simulink model "sschdlexThreePhaseTwoLevelInverterModel"  (R2026a)
settings: Solver=FixedStepDiscrete  StopTime=0.05
undefined symbols (not defined in the file or in its folder): ee_sli_rtmsupport, gcbh
libraries: fl_lib x17, nesl_utility x17, ee_lib x9
settings Model: DataTypeOverride=Off  Creator=The MathWorks, Inc.  LastModifiedBy=The MathWorks, Inc.
settings OptimizationCC: ConditionallyExecuteInputs=off  InheritOutputTypeSmallerThanSingle=on
settings DebuggingCC: ArtificialAlgebraicLoopMsg=error  SingleTaskRateTransMsg=error
settings HardwareCC: ProdHWDeviceType=ASIC/FPGA->ASIC/FPGA  TargetBitPerLong=64.0  TargetBitPerPointer=64.0  TargetBitPerSizeT=64.0  TargetBitPerPtrDiffT=64.0  TargetLongLongMode=on  TargetIntDivRoundTo=Zero  TargetEndianess=LittleEndian  TargetWordSize=64.0  TargetHWDeviceType=Custom Processor->MATLAB Host Computer  ProdEqTarget=off
settings SimscapeCC: SimscapeNominalValues="[{\"value\":\"1\",\"unit\":\"A\"},{\"value\":\"1\",\"unit\":\"bar\"},{\"value\":\"1\",\"unit\":\"cm^2\"},{\"value\":\"1\",\"unit\":\"cm^3/s\"},{\"value\":\"1\",\"unit\":\"kJ/kg\"},{\"value\":\"1\",\"unit\":\"kW\"},{\"value\":\"1\",\"unit\":\"l\"},{\"value\":\"1\",\"unit\":\"N\"},{\"value\":\"1\",\"unit\":\"N*m\"},{\"value\":\"1\",\"unit\":\"V\"}]"  SimscapeLogType=none  SimscapeLogDataHistory=5000.0

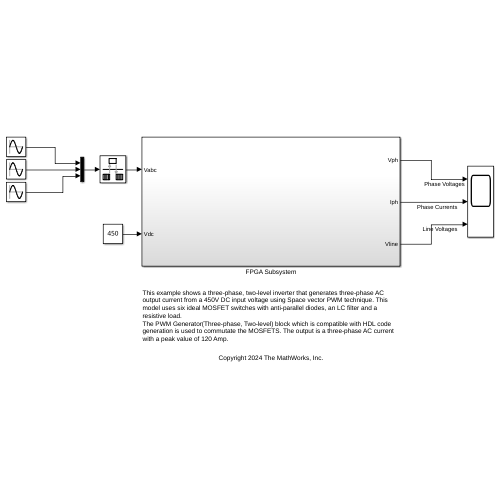
[thumbnail: Simulink's stored preview of the top-level diagram]
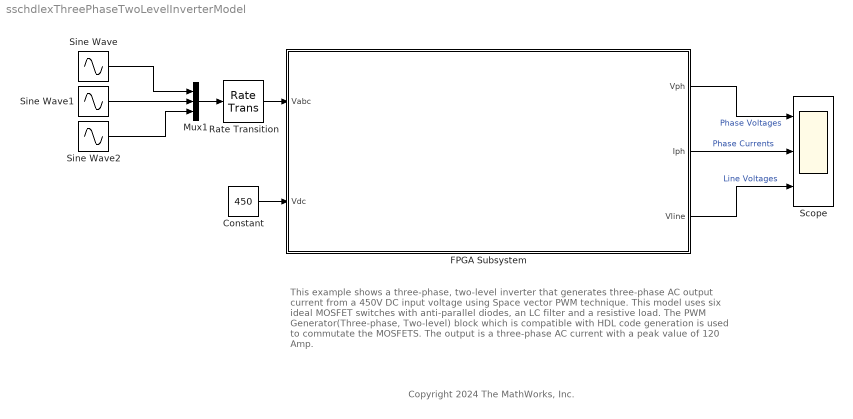
== system sschdlexThreePhaseTwoLevelInverterModel ==
  note: This example shows a three-phase, two-level inverter that generates three-phase AC output current from a 450V DC input voltage using Space vector PWM technique. This model uses six ideal MOSFET switches with anti-parallel diodes, an LC filter and a resistive load.
      | The PWM Generator(Three-phase, Two-level) block which is compatible with HDL code generation is used to commutate the MOSFETS. The output is a three-phase AC current with a peak value of 120 Amp.
  note: Copyright 2024 The MathWorks, Inc.
  Constant : Constant  Value=450  SampleTime=-1
  FPGA Subsystem : Subsystem
  Mux1 : Mux  Inputs=3
  Rate Transition : RateTransition
  Scope : Scope  NumInputPorts=3
      settings: ActiveDisplayYMinimum=159.51111  ActiveDisplayYMaximum=229.40651
  Sine Wave : Sin  Amplitude=200  Frequency=2*pi*50  SampleTime=0
  Sine Wave1 : Sin  Amplitude=200  Frequency=2*pi*50  Phase=-2*pi/3  SampleTime=0
  Sine Wave2 : Sin  Amplitude=200  Frequency=2*pi*50  Phase=-4*pi/3  SampleTime=0
  wires:
  Sine Wave/1 -> Mux1/1
  Sine Wave1/1 -> Mux1/2
  Sine Wave2/1 -> Mux1/3
  Mux1/1 -> Rate Transition/1
  FPGA Subsystem/3(Vline) -> Scope/3  "Line Voltages"
  FPGA Subsystem/1(Vph) -> Scope/1  "Phase Voltages"
  FPGA Subsystem/2(Iph) -> Scope/2  "Phase Currents"
  Rate Transition/1 -> FPGA Subsystem/1(Vabc)
  Constant/1 -> FPGA Subsystem/2(Vdc)

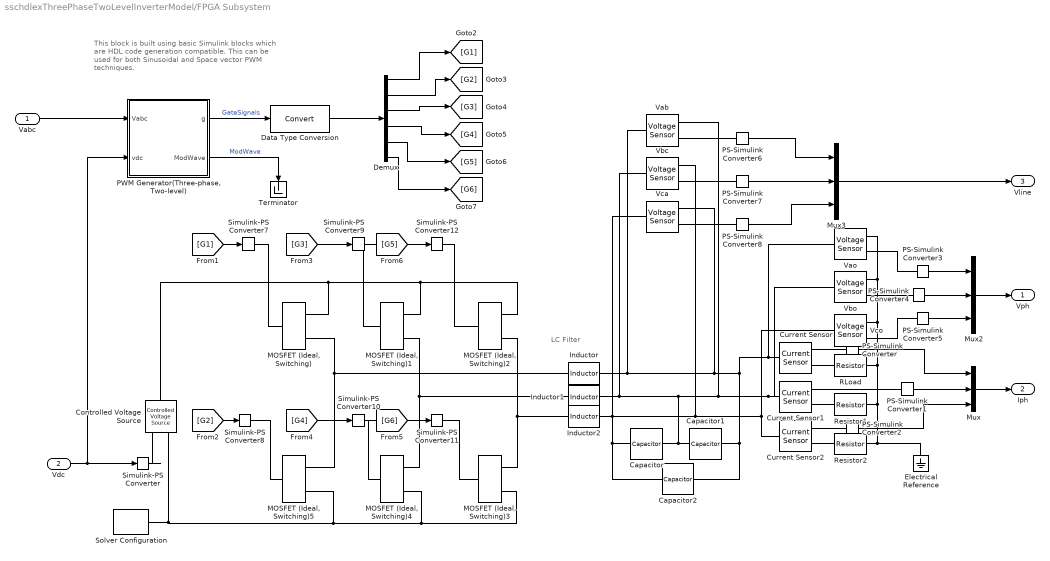
== system sschdlexThreePhaseTwoLevelInverterModel/FPGA Subsystem ==
  note: This block is built using basic Simulink
      | blocks which are HDL code generation
      | compatible. This can be used for both
      | Sinusoidal and Space vector PWM
      | techniques.
  note: LC Filter
  Vabc : Inport
  Vdc : Inport  Port=2
  Capacitor : fl_lib/Electrical/Electrical Elements/Capacitor  c=470e-6 F  r=1e9 Ohm  g=0 1/Ohm  i_specify=off  i_priority=None  i=0 A  i_nominal_specify=off  i_nominal_value=1  i_nominal_unit=A  v_specify=off  v_priority=None  v=0 V  v_nominal_specify=off  v_nominal_value=1  v_nominal_unit=V  vc_specify=off  vc_priority=High  vc=0 V  vc_nominal_specify=off  vc_nominal_value=1  vc_nominal_unit=V
  Capacitor1 : fl_lib/Electrical/Electrical Elements/Capacitor  c=470e-6 F  r=1e9 Ohm  g=0 1/Ohm  i_specify=off  i_priority=None  i=0 A  i_nominal_specify=off  i_nominal_value=1  i_nominal_unit=A  v_specify=off  v_priority=None  v=0 V  v_nominal_specify=off  v_nominal_value=1  v_nominal_unit=V  vc_specify=off  vc_priority=High  vc=0 V  vc_nominal_specify=off  vc_nominal_value=1  vc_nominal_unit=V
  Capacitor2 : fl_lib/Electrical/Electrical Elements/Capacitor  c=470e-6 F  r=1e9 Ohm  g=0 1/Ohm  i_specify=off  i_priority=None  i=0 A  i_nominal_specify=off  i_nominal_value=1  i_nominal_unit=A  v_specify=off  v_priority=None  v=0 V  v_nominal_specify=off  v_nominal_value=1  v_nominal_unit=V  vc_specify=off  vc_priority=High  vc=0 V  vc_nominal_specify=off  vc_nominal_value=1  vc_nominal_unit=V
  Controlled Voltage Source : fl_lib/Electrical/Electrical Sources/Controlled Voltage Source
  Current Sensor : fl_lib/Electrical/Electrical Sensors/Current Sensor
  Current Sensor1 : fl_lib/Electrical/Electrical Sensors/Current Sensor
  Current Sensor2 : fl_lib/Electrical/Electrical Sensors/Current Sensor
  Data Type Conversion : DataTypeConversion  SaturateOnIntegerOverflow=off  RndMeth=Floor
  Demux : Demux  Outputs=6
  Electrical Reference : fl_lib/Electrical/Electrical Elements/Electrical Reference
  Inductor : ee_lib/Passive/Inductor  l=350e-6 H  enable_L_tol=ee.enum.toleranceApplication.none  L_tol=20  tol_distribution=ee.enum.toleranceDistribution.uniform  nSigma=4  r=0 Ohm  g=1e-9 1/Ohm  enable_operating_limits=ee.enum.enable.no  operating_limit_action=ee.enum.passive.reportOpLim.warn  max_working_current=1 A  power_rating=1 W  i_L_specify=off  i_L_priority=High  i_L=0 A  i_L_nominal_specify=off  i_L_nominal_value=1  i_L_nominal_unit=A
  Inductor1 : ee_lib/Passive/Inductor  l=350e-6 H  enable_L_tol=ee.enum.toleranceApplication.none  L_tol=20  tol_distribution=ee.enum.toleranceDistribution.uniform  nSigma=4  r=0 Ohm  g=1e-9 1/Ohm  enable_operating_limits=ee.enum.enable.no  operating_limit_action=ee.enum.passive.reportOpLim.warn  max_working_current=1 A  power_rating=1 W  i_L_specify=off  i_L_priority=High  i_L=0 A  i_L_nominal_specify=off  i_L_nominal_value=1  i_L_nominal_unit=A
  Inductor2 : ee_lib/Passive/Inductor  l=350e-6 H  enable_L_tol=ee.enum.toleranceApplication.none  L_tol=20  tol_distribution=ee.enum.toleranceDistribution.uniform  nSigma=4  r=0 Ohm  g=1e-9 1/Ohm  enable_operating_limits=ee.enum.enable.no  operating_limit_action=ee.enum.passive.reportOpLim.warn  max_working_current=1 A  power_rating=1 W  i_L_specify=off  i_L_priority=High  i_L=0 A  i_L_nominal_specify=off  i_L_nominal_value=1  i_L_nominal_unit=A
  MOSFET (Ideal, Switching){,1..5} (6 alike) : ee_lib/Semiconductors & Converters/MOSFET (Ideal, Switching)  port_option=ee.enum.controlport.ps  Rds=0.001 Ohm  Goff=1e-6 1/Ohm  Vth=0.5 V  diode_param=2  diode_Vf=0.8 V  diode_Ron=0.001 Ohm  diode_Goff=1e-5 1/Ohm  diode_C=50e-9 F  diode_iRM=-235 A  diode_iF=300 A  diode_idot=-50 A/us  diode_trr_param=1  diode_trr_factor=3  diode_trr=15 us  diode_Qrr=1500 s*uA  ids_specify=off  ids_priority=None  ids=0 A  ids_nominal_specify=off  ids_nominal_value=1  ids_nominal_unit=A  vds_specify=off  vds_priority=None  vds=0 V  vds_nominal_specify=off  vds_nominal_value=1  vds_nominal_unit=V  vgs_specify=off  vgs_priority=None  vgs=0 V  vgs_nominal_specify=off  vgs_nominal_value=1  vgs_nominal_unit=V  thermal_loss_option=ee.enum.converters.thermalLossOption.constantvalues  Von_data=[0, 1.8, 3.2, 6, 10, 16; 0, 2, 5.5, 9.5, 15, 25] V  Tj=[298.15, 448.15] K  Iout_data=[0, 20, 40, 60, 80, 100] A  tabulateWithVds=false  Eon_data=[0, 55.04, 124.57, 235.53, 362.12; 0, 71.25, 161.25, 304.88, 468.75] * 1e-6 J  Eoff_data=[0, 18, 30, 56.1, 76.5; 0, 22.5, 37.5, 70.13, 95.63] * 1e-6 J  Eon_data_3D=[zeros(2, 5, 3)] J  Eoff_data_3D=[zeros(2, 5, 3)] J  Tj_loss=[298.15, 448.15] K  Iout_data_loss=[0, 10, 20, 30, 40] A  Vds_loss=[0, 150, 300] V  Eon_scalar=22.86e-3 J  Eoff_scalar=17.14e-3 J  Voff=300 V  Iout_scalar=600 A  useCurrentFromPreviousCycle=false  useVoltageFromPreviousCycle=false  diodeModelType=ee.enum.converters.diodeModelType.pwl  diodeTableType=ee.enum.diode.tableType.IfMat  diode_ReverseIVType=ee.enum.diode.diodeReverseIV.constant  diode_IfMat=[.07, .12, .19, 1.75, 4.24, 7.32, 11.2; .16, .3, .72, 2.14, 4.02, 6.35, 9.12] A  diode_VfMat=[.9, 1.15, 1.25, 1.5, 1.75, 2.17, 2.6, 2.85; .58, .68, .75, 1.1, 1.38, 1.77, 2.27, 2.7] V  diode_TjVec=[25, 125] degC  diode_VfVec=[.5, .7, .9, 1.3, 1.7, 2.1, 2.5] V  diode_IfVec=[.1, .2, .5, 1, 2, 4, 7, 10] A  diode_IrMat=[1e-06, 2e-06, 5e-06, 1e-05, 2.5e-05, 5e-05, .0001; 2e-06, 5e-06, 1e-05, 4e-05, 8e-05, .0002, .0005] A  diode_VrMat=[10, 100, 200, 250, 300, 325, 350; 10, 70, 160, 220, 270, 300, 320] V  diode_VrVec=[10, 20, 40, 50, 70, 80, 100] V  diode_IrVec=[1e-06, 2e-06, 5e-06, 1e-05, 2e-05, 5e-05, .0001] A  diode_Vr=-600 V  diode_Ls=150 nH  diode_Erec=0.03 J  diode_rec_loss_model=ee.enum.diode.reverseRecoveryModel.fixed  diode_ErecVal=0 J  diode_scaleWithIandV=true  diode_ErecMat=zeros(2, 3) J  diodeErecMat3D=zeros(2, 3, 2) J  diode_TjrecVec=[298.15, 398.15] K  diode_IfrecVec=[.1, 1, 10] A  diodeVrecVec=[0, 100] V  diode_IrecVal=10 A  diode_VrecVal=10 V  diode_tFilter=1 / 1000 / 100 s  separateThermalPortForDiode=false  thermal_network_parameterization=ee.enum.thermalNetworkTopology.external  Rth=[.03, .2] K/W  Rth_Cauer=[.03, .1, .2] K/W  Rth_Foster=[.03, .2] K/W  thermal_mass_parameterization=ee.enum.thermalNetwork.timeconstant  thermal_mass=[3, 25] J/K  thermal_mass_Cauer=[3, 10, 25] J/K  thermal_mass_Foster=[33, 50] J/K  thermal_time_constant=[.1, 5] s  thermal_time_constant_Cauer=[.1, 1, 5] s  thermal_time_constant_Foster=[1, 10] s  thermal_mass_initial_temperatures=[25, 25] degC  thermal_mass_initial_temperatures_Cauer=[25, 25, 25] degC  junction_thermal_mass=0.1 J/K  Tvec_initial_Foster=[25, 25, 25, 25] degC  RthDiode=[.03, .2] K/W  RthCauerDiode=[.03, .1, .2] K/W  RthFosterDiode=[.03, .2] K/W  thermalMassDiode=[3, 25] J/K  thermalMassCauerDiode=[3, 10, 25] J/K  thermalMassFosterDiode=[33, 50] J/K  thermalTauDiode=[.1, 5] s  thermalTauCauerDiode=[.1, 1, 5] s  thermalTauFosterDiode=[1, 10] s  thermalMassInitTempDiode=[25, 25] degC  thermalMassInitTempCauerDiode=[25, 25, 25] degC  junctionthermalMassDiode=0.1 J/K  TVecInitialFosterDiode=[25, 25, 25, 25] degC  no_thermal_network=0  mosfet_junction_temperature_specify=off  mosfet_junction_temperature_priority=None  mosfet_junction_temperature=25 degC  mosfet_junction_temperature_nominal_specify=off  mosfet_junction_temperature_nominal_value=1  mosfet_junction_temperature_nominal_unit=degC  diode_junction_temperature_specify=off  diode_junction_temperature_priority=None  diode_junction_temperature=25 degC  diode_junction_temperature_nominal_specify=off  diode_junction_temperature_nominal_value=1  diode_junction_temperature_nominal_unit=degC  Qj_specify=off  Qj_priority=None  Qj=0 W  Qj_nominal_specify=off  Qj_nominal_value=1  Qj_nominal_unit=W  accumulatedSwitchingLosses_specify=off  accumulatedSwitchingLosses_priority=None  accumulatedSwitchingLosses=0 J
  Mux : Mux  Inputs=3
  Mux2 : Mux  Inputs=3
  Mux3 : Mux  Inputs=3
  PS-Simulink Converter{,1..8} (9 alike) : nesl_utility/PS-Simulink Converter  PhysicalDomain=network_engine_domain  SubClassName=ps_output  LeftPortType=input  RightPortType=output  PseudoPeriodic=off  Frequencies=[]  VectorFormat=inherit  Unit=inherit  AffineConversion=off
  "PWM Generator(Three-phase, Two-level)" : Subsystem  LoadFcn=ee_sli_rtmsupport( 'loadfcn', gcbh );  mask(PWM Generator (three-phase, two-level)){PWMMode=Continuous PWM (CPWM), CPWMMode=SVM: space vector modulation, DPWMMode=60 DPWM: 60 degree discontinuous PWM, SamplingMode=Natural, fsw=15e3, Ts=1e-6}
      mask prompts: PWMMode "physmod:ee:library:comments:control:eePwmGeneratorTwoLevel:PWMMode_MP"; CPWMMode "physmod:ee:library:comments:control:eePwmGeneratorTwoLevel:ContinuousPWM_MP"; DPWMMode "physmod:ee:library:comments:control:eePwmGeneratorTwoLevel:DiscontinuousPWM_MP"; SamplingMode "physmod:ee:library:comments:control:eePwmGeneratorTwoLevel:SamplingMode_MP"; fsw "physmod:ee:library:comments:control:eePwmGeneratorTwoLevel:SwitchingFrequencyHz_MP"; Ts "physmod:ee:library:comments:control:eePwmGeneratorTwoLevel:SampleTimes_MP"
      mask help: physmod:ee:library:comments:control:eePwmGeneratorTwoLevel:PWMGeneratorthreephaseTwolevel_MD
      mask init:
      | Tsw = 1/fsw;
      | 
      | if fsw <= 0
      |     error(message('physmod:simscape:compiler:patterns:checks:GreaterThanZero',getString(message('physmod:ee:library:comments:control:eePwmGeneratorTwoLevel:SwitchingFrequencyHz_MP'))));
      | end
      | 
      | if Ts <= 0
      |     error(message('physmod:simscape:compiler:patterns:checks:GreaterThanZero',getString(message('physmod:ee:library:comments:control:eePwmGeneratorTwoLevel:SampleTimes_MP'))));
      | end
      | 
      | if Ts > 1/(10*fsw)
      |     error(message('physmod:simscape:compiler:patterns:checks:LessThanOrEqual',getString(message('physmod:ee:library:comments:control:eePwmGeneratorTwoLevel:SampleTimes_MP')),getString(message('physmod:ee:library:comments:control:eePwmGeneratorTwoLevel:inverseOf10TimesSwitchingFrequency_MP'))));
      | end
      | 
      | switch SamplingMode
      |     case 'Natural'
      |         RateTransitionOnInput = -1;
      |         GateGeneratorX0 = 0;
      |     case 'Asymmetric'
      |         RateTransitionOnInput = 0.5*Tsw;
      |         GateGeneratorX0 = 0.5/fsw;
      |     case 'Symmetric'
      |         RateTransitionOnInput = Tsw;
      |         GateGeneratorX0 = 0;
      | end
      | 
      | 
      | switch PWMMode
      |     case 'Continuous PWM (CPWM)'
      |         switch CPWMMode
      |             case 'SPWM: sinusoidal PWM'
      |                 PWM = 1;
      |             case 'SVM: space vector modulation'
      |                 PWM = 2;
      |         end
      |     case 'Discontinuous PWM (DPWM)'
      |         switch DPWMMode
      |             case '60 DPWM: 60 degree discontinuous PWM'
      |                 PWM = 3;
      |             case '60 DPWM (+30 degree shift): +30 degree shift from 60 DPWM'
      |                 PWM = 4;
      |             case '60 DPWM (-30 degree shift): -30 degree shift from 60 DPWM'
      |                 PWM = 5;
      |             case '30 DPWM: 30 degree discontinuous PWM'
      |                 PWM = 6;
      |             case '120 DPWM: positive dc component'
      |                 PWM = 7;
      |             case '120 DPWM: negative dc component'
      |                 PWM = 8;
      |         end
      | end
      settings: CopyFcn=ee_sli_rtmsupport( 'copyfcn', gcbh );  DeleteFcn=ee_sli_rtmsupport( 'deletefcn', gcbh );  ModelCloseFcn=ee_sli_rtmsupport( 'modelclosefcn', gcbh );  PreSaveFcn=%pe_sli_rtmsupport( 'presavefcn', gcbh );  PostSaveFcn=ee_sli_rtmsupport( 'postsavefcn', gcbh );  PreCopyFcn=ee_sli_rtmsupport( 'precopyfcn', gcbh );  OpenFcn=ee_sli_rtmsupport( 'openfcn', gcbh );  CloseFcn=ee_sli_rtmsupport( 'closefcn', gcbh );  PreDeleteFcn=ee_sli_rtmsupport( 'predeletefcn', gcbh );
      settings: LibrarySourceBlock=|
      | eePwmGeneratorTwoLevel/PWM Generator
      | (Three-phase, Two-level)
      mask Help: web(nesl_help(gcbh))
      mask TypeOptions PWMMode: physmod:ee:library:comments:control:eePwmGeneratorTwoLevel:ContinuousPWMCPWM_PV | physmod:ee:library:comments:control:eePwmGeneratorTwoLevel:DiscontinuousPWMDPWM_PV
      mask Callback PWMMode:
      | switch get_param(gcb,'PWMMode')
      |     case 'Continuous PWM (CPWM)'
      |         set_param(gcb,'MaskVisibilities',{'on';'on';'off';'on';'on';'on'})
      |     case 'Discontinuous PWM (DPWM)'
      |         set_param(gcb,'MaskVisibilities',{'on';'off';'on';'on';'on';'on'})
      | end
      mask TypeOptions CPWMMode: physmod:ee:library:comments:control:eePwmGeneratorTwoLevel:SPWMSinusoidalPWM_PV | physmod:ee:library:comments:control:eePwmGeneratorTwoLevel:SVMSpaceVectorModulation_PV
      mask TypeOptions DPWMMode: physmod:ee:library:comments:control:eePwmGeneratorTwoLevel:x60DPWM60DegreeDiscontinuousPWM_PV | physmod:ee:library:comments:control:eePwmGeneratorTwoLevel:x60DPWM30DegreeShift30DegreeShiftFrom60DPWM_PV | physmod:ee:library:comments:control:eePwmGeneratorTwoLevel:x60DPWM0x2D30DegreeShift0x2D30DegreeShiftFrom60DPWM_PV | physmod:ee:library:comments:control:eePwmGeneratorTwoLevel:x30DPWM30DegreeDiscontinuousPWM_PV | physmod:ee:library:comments:control:eePwmGeneratorTwoLevel:x120DPWMPositiveDcComponent_PV | physmod:ee:library:comments:control:eePwmGeneratorTwoLevel:x120DPWMNegativeDcComponent_PV
      mask TypeOptions SamplingMode: physmod:ee:library:comments:control:eePwmGeneratorTwoLevel:Natural_PV | physmod:ee:library:comments:control:eePwmGeneratorTwoLevel:Asymmetric_PV | physmod:ee:library:comments:control:eePwmGeneratorTwoLevel:Symmetric_PV
      mask DialogControl ParameterGroupVar Prompt: physmod:ee:library:comments:control:eePwmGeneratorTwoLevel:tab_Parameters
      mask DialogControl PWMMode Prompt: PWM mode
      mask DialogControl CPWMMode Prompt: Continuous PWM
      mask DialogControl DPWMMode Prompt: Discontinuous PWM
      mask DialogControl SamplingMode Prompt: Sampling mode
      mask DialogControl fsw Prompt: Switching frequency (Hz)
      mask DialogControl Ts Prompt: Sample time (s)
  RLoad : fl_lib/Electrical/Electrical Elements/Resistor  R=1.65 Ohm  i_specify=off  i_priority=None  i=0 A  i_nominal_specify=off  i_nominal_value=1  i_nominal_unit=A  v_specify=off  v_priority=None  v=0 V  v_nominal_specify=off  v_nominal_value=1  v_nominal_unit=V
  Resistor1 : fl_lib/Electrical/Electrical Elements/Resistor  R=1.65 Ohm  i_specify=off  i_priority=None  i=0 A  i_nominal_specify=off  i_nominal_value=1  i_nominal_unit=A  v_specify=off  v_priority=None  v=0 V  v_nominal_specify=off  v_nominal_value=1  v_nominal_unit=V
  Resistor2 : fl_lib/Electrical/Electrical Elements/Resistor  R=1.65 Ohm  i_specify=off  i_priority=None  i=0 A  i_nominal_specify=off  i_nominal_value=1  i_nominal_unit=A  v_specify=off  v_priority=None  v=0 V  v_nominal_specify=off  v_nominal_value=1  v_nominal_unit=V
  Simulink-PS Converter{,7..12} (7 alike) : nesl_utility/Simulink-PS Converter  PhysicalDomain=network_engine_domain  SubClassName=ps_input  LeftPortType=input  RightPortType=output  PseudoPeriodic=off  Frequencies=[]  NoiseDistribution=none  NoiseParameters=[]  Unit=1  AffineConversion=off  FilteringAndDerivatives=provide  SimscapeFilterOrder=1  InputFilterTimeConstant=0.001  UdotUserProvided=0
  Solver Configuration : nesl_utility/Solver Configuration  PhysicalDomain=network_engine_domain  SubClassName=solver  LeftPortType=input  RightPortType=generic  Tones=[]  Harmonics=[]  SimulateNoise=off  Profile=off  UseLocalSampling=off  EnableSwitchedLinearOptims=on  FrequencyDomain=off  UseCCode=off  RelTol=0.001  AbsTol=0.001  MinStep=1e-09  ToWorkspace=off  RevertToSquareIcSolve=off  NumHomotopyIterations=100  PhasorMode=off  PhasorModeNumHarmonics=1  ConsistencySolver=NEWTON_XTOL_AFTER_FTOL  CanonicalOrdering=UNORDERED  OptimizeIntermediates=UNOPTIMIZED  IndexReductionMethod=DerivativeReplacement  DoDC=off  ResidualTolerance=1e-09  ConsistencyTolSource=GLOBAL  ConsistencyAbsTol=0.001  ConsistencyRelTol=0.001  ConsistencyTolFactor=0.001  UseLocalSolver=on  LocalSolverChoice=NE_BACKWARD_EULER_ADVANCER  ResolveIndetEquations=on  FunctionEvalNumThread=1  LocalSolverSampleTime=1e-6  DoFixedCost=off  MaxNonlinIter=3  MaxModeIter=2  ComputeImpulses=off  ImpulseIterations=2  LinearAlgebra=auto  LinearAlgebraNumThread=0  EquationFormulation=NE_TIME_EF  DelaysMemoryBudget=1024  AutomaticFiltering=on  FilteringTimeConstant=0.001  PartitionStorageMethod=AS_NEEDED  PartitionMemoryBudget=1024  PartitionMethod=ROBUST  MultibodyUseLocalSolver=off  MultibodyLocalSolverChoice=ODE1  MultibodyLocalSolverSampleTime=0.001
  Terminator : Terminator
  Vab : fl_lib/Electrical/Electrical Sensors/Voltage Sensor
  Vao : fl_lib/Electrical/Electrical Sensors/Voltage Sensor
  Vbc : fl_lib/Electrical/Electrical Sensors/Voltage Sensor
  Vbo : fl_lib/Electrical/Electrical Sensors/Voltage Sensor
  Vca : fl_lib/Electrical/Electrical Sensors/Voltage Sensor
  Vco : fl_lib/Electrical/Electrical Sensors/Voltage Sensor
  Vph : Outport
  Iph : Outport  Port=2
  Vline : Outport  Port=3
  wires:
  Demux/2 -> [G2]
  [G5] -> Simulink-PS Converter12/1
  PS-Simulink Converter5/1 -> Mux2/3
  PS-Simulink Converter/1 -> Mux/1
  [G1] -> Simulink-PS Converter7/1
  [G4] -> Simulink-PS Converter10/1
  Demux/3 -> [G3]
  PS-Simulink Converter1/1 -> Mux/2
  Mux/1 -> Iph/1
  Vdc/1 -> Simulink-PS Converter/1, "PWM Generator(Three-phase, Two-level)"/2(vdc)
  [G2] -> Simulink-PS Converter8/1
  PS-Simulink Converter3/1 -> Mux2/1
  Demux/1 -> [G1]
  Data Type Conversion/1 -> Demux/1
  Demux/4 -> [G4]
  Demux/6 -> [G6]
  Demux/5 -> [G5]
  PS-Simulink Converter2/1 -> Mux/3
  [G3] -> Simulink-PS Converter9/1
  "PWM Generator(Three-phase, Two-level)"/1(g) -> Data Type Conversion/1  "GateSignals"
  Mux3/1 -> Vline/1
  PS-Simulink Converter4/1 -> Mux2/2
  Mux2/1 -> Vph/1
  [G6] -> Simulink-PS Converter11/1
  "PWM Generator(Three-phase, Two-level)"/2(ModWave) -> Terminator/1  "ModWave"
  Vabc/1 -> "PWM Generator(Three-phase, Two-level)"/1(Vabc)
  PS-Simulink Converter6/1 -> Mux3/1
  PS-Simulink Converter7/1 -> Mux3/2
  PS-Simulink Converter8/1 -> Mux3/3
  connections:
  Inductor/LConn1 -- "MOSFET (Ideal, Switching)5"/RConn1 -- "MOSFET (Ideal, Switching)"/RConn2
  "MOSFET (Ideal, Switching)2"/RConn1 -- "MOSFET (Ideal, Switching)1"/RConn1 -- "MOSFET (Ideal, Switching)"/RConn1 -- Controlled Voltage Source/LConn1
  Capacitor/LConn1 -- Vco/LConn1 -- Current Sensor2/LConn1 -- Vbc/RConn2 -- Vca/LConn1 -- Inductor2/RConn1 -- Capacitor2/LConn1
  RLoad/LConn1 -- Current Sensor/RConn2
  Resistor2/RConn1 -- Vao/RConn2 -- Vbo/RConn2 -- Vco/RConn2 -- RLoad/RConn1 -- Resistor1/RConn1 -- Electrical Reference/LConn1
  Inductor1/LConn1 -- "MOSFET (Ideal, Switching)4"/RConn1 -- "MOSFET (Ideal, Switching)1"/RConn2
  "MOSFET (Ideal, Switching)3"/RConn2 -- "MOSFET (Ideal, Switching)4"/RConn2 -- "MOSFET (Ideal, Switching)5"/RConn2 -- Solver Configuration/RConn1 -- Controlled Voltage Source/RConn2
  Resistor1/LConn1 -- Current Sensor1/RConn2
  Simulink-PS Converter10/RConn1 -- "MOSFET (Ideal, Switching)4"/LConn1
  Resistor2/LConn1 -- Current Sensor2/RConn2
  Capacitor/RConn1 -- Inductor1/RConn1 -- Vbc/LConn1 -- Vbo/LConn1 -- Current Sensor1/LConn1 -- Vab/RConn2 -- Capacitor1/LConn1
  Vab/RConn1 -- PS-Simulink Converter6/LConn1
  Capacitor1/RConn1 -- Inductor/RConn1 -- Vab/LConn1 -- Vca/RConn2 -- Vao/LConn1 -- Current Sensor/LConn1 -- Capacitor2/RConn1
  Simulink-PS Converter/RConn1 -- Controlled Voltage Source/RConn1
  Simulink-PS Converter12/RConn1 -- "MOSFET (Ideal, Switching)2"/LConn1
  PS-Simulink Converter3/LConn1 -- Vao/RConn1
  PS-Simulink Converter1/LConn1 -- Current Sensor1/RConn1
  Vca/RConn1 -- PS-Simulink Converter8/LConn1
  Inductor2/LConn1 -- "MOSFET (Ideal, Switching)3"/RConn1 -- "MOSFET (Ideal, Switching)2"/RConn2
  Simulink-PS Converter9/RConn1 -- "MOSFET (Ideal, Switching)1"/LConn1
  Simulink-PS Converter7/RConn1 -- "MOSFET (Ideal, Switching)"/LConn1
  PS-Simulink Converter2/LConn1 -- Current Sensor2/RConn1
  Vbo/RConn1 -- PS-Simulink Converter4/LConn1
  PS-Simulink Converter/LConn1 -- Current Sensor/RConn1
  Simulink-PS Converter11/RConn1 -- "MOSFET (Ideal, Switching)3"/LConn1
  PS-Simulink Converter7/LConn1 -- Vbc/RConn1
  Simulink-PS Converter8/RConn1 -- "MOSFET (Ideal, Switching)5"/LConn1
  Vco/RConn1 -- PS-Simulink Converter5/LConn1

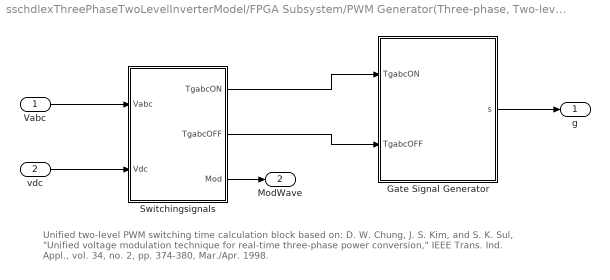
== system sschdlexThreePhaseTwoLevelInverterModel/FPGA Subsystem/PWM Generator(Three-phase, Two-level) ==
  note: Unified two-level PWM switching time calculation block based on:
      | D. W. Chung, J. S. Kim, and S. K. Sul, "Unified voltage modulation technique for real-time three-phase power conversion," IEEE Trans. Ind. Appl., vol. 34, no. 2, pp. 374-380, Mar./Apr. 1998.
  Vabc : Inport
  vdc : Inport  Port=2
  Gate Signal Generator : Subsystem
      settings: LibrarySourceBlock=|
      | eePwmGeneratorTwoLevel/PWM Generator
      | (Three-phase, Two-level)/Gate Signal
      | Generator
  Switchingsignals : Subsystem
  g : Outport  VectorParamsAs1DForOutWhenUnconnected=off
  ModWave : Outport  Port=2  VectorParamsAs1DForOutWhenUnconnected=off
  wires:
  vdc/1 -> Switchingsignals/2(Vdc)
  Vabc/1 -> Switchingsignals/1(Vabc)
  Gate Signal Generator/1(s) -> g/1
  Switchingsignals/3(Mod) -> ModWave/1
  Switchingsignals/2(TgabcOFF) -> Gate Signal Generator/2(TgabcOFF)
  Switchingsignals/1(TgabcON) -> Gate Signal Generator/1(TgabcON)

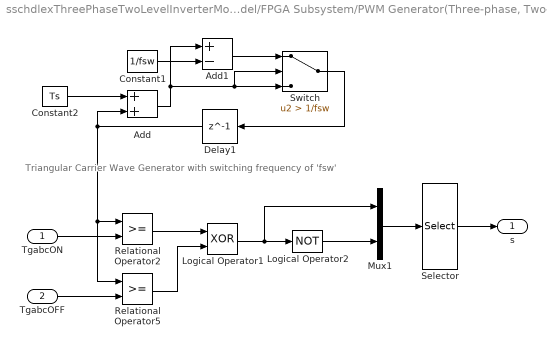
== system sschdlexThreePhaseTwoLevelInverterModel/FPGA Subsystem/PWM Generator(Three-phase, Two-level)/Gate Signal Generator ==
  note: Triangular Carrier Wave Generator with switching frequency of 'fsw'
  TgabcON : Inport
  TgabcOFF : Inport  Port=2
  Add : Sum
  Add1 : Sum  Inputs=+-
  Constant1 : Constant  Value=1/fsw
  Constant2 : Constant  Value=Ts
  Delay1 : Delay  DelayLength=1  InitialCondition=GateGeneratorX0  SampleTime=Ts
  Logical Operator1 : Logic  Operator=XOR  AllPortsSameDT=off  OutDataTypeStr=boolean
  Logical Operator2 : Logic  Operator=NOT  AllPortsSameDT=off  OutDataTypeStr=boolean
  Mux1 : Mux  Inputs=2
  Relational Operator2 : RelationalOperator  OutDataTypeStr=boolean  InputSameDT=off
  Relational Operator5 : RelationalOperator  OutDataTypeStr=boolean  InputSameDT=off
  Selector : Selector  InputPortWidth=6  IndexOptions=Index vector (dialog)  Indices=[1 4 2 5 3 6]  OutputSizes=1
  Switch : Switch  Criteria=u2 > Threshold  Threshold=1/fsw  SaturateOnIntegerOverflow=off  InputSameDT=off
  s : Outport  VectorParamsAs1DForOutWhenUnconnected=off
  wires:
  Delay1/1 -> Add/2, Relational Operator2/1, Relational Operator5/1
  Constant2/1 -> Add/1
  Relational Operator2/1 -> Logical Operator1/1
  TgabcON/1 -> Relational Operator2/2
  Relational Operator5/1 -> Logical Operator1/2
  Add/1 -> Switch/2, Switch/3, Add1/1
  Switch/1 -> Delay1/1
  TgabcOFF/1 -> Relational Operator5/2
  Constant1/1 -> Add1/2
  Add1/1 -> Switch/1
  Logical Operator1/1 -> Mux1/1, Logical Operator2/1
  Selector/1 -> s/1
  Mux1/1 -> Selector/1
  Logical Operator2/1 -> Mux1/2

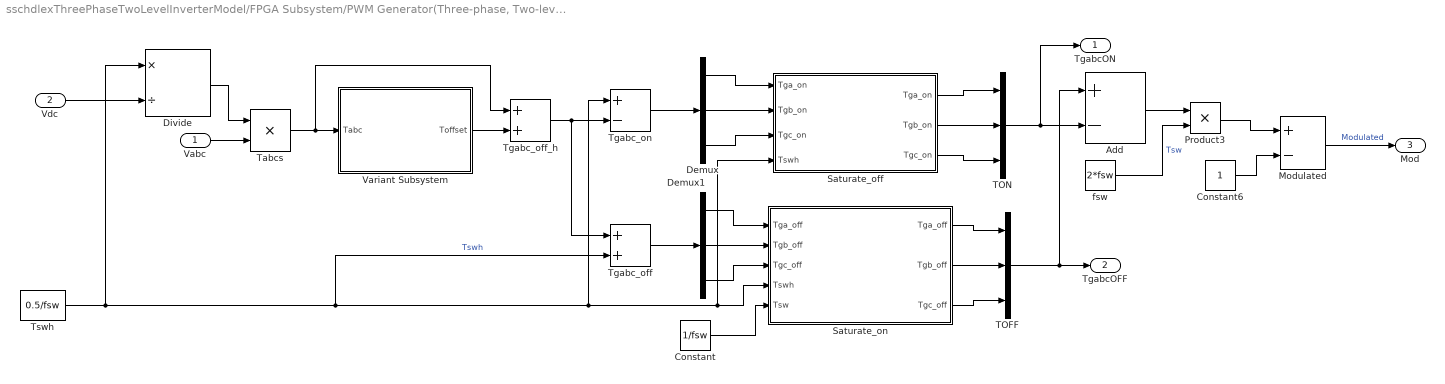
== system sschdlexThreePhaseTwoLevelInverterModel/FPGA Subsystem/PWM Generator(Three-phase, Two-level)/Switchingsignals ==
  Vabc : Inport
  Vdc : Inport  Port=2
  Add : Sum  Inputs=+-
  Constant : Constant  Value=1/fsw  SampleTime=-1
  Constant6 : Constant  SampleTime=-1
  Demux : Demux  Outputs=3
  Demux1 : Demux  Outputs=3
  Divide : Product  Inputs=*/
  Modulated : Sum  Inputs=+-
  Product3 : Product
  Saturate_off : MATLAB Function  TreatAsAtomicUnit=on
  Saturate_on : MATLAB Function  TreatAsAtomicUnit=on
  TOFF : Mux  Inputs=3
  TON : Mux  Inputs=3
  Tabcs : Product
  Tgabc_off : Sum
  Tgabc_off_h : Sum
  Tgabc_on : Sum  Inputs=+-
  Tswh : Constant  Value=0.5/fsw
  Variant Subsystem : Subsystem  Variant=on
  fsw : Constant  Value=2*fsw
  TgabcON : Outport  VectorParamsAs1DForOutWhenUnconnected=off
  TgabcOFF : Outport  Port=2  VectorParamsAs1DForOutWhenUnconnected=off
  Mod : Outport  Port=3  VectorParamsAs1DForOutWhenUnconnected=off
  wires:
  Variant Subsystem/1(Toffset) -> Tgabc_off_h/2
  Vabc/1 -> Tabcs/2
  Vdc/1 -> Divide/2
  Tswh/1 -> Saturate_off/4(Tswh), Saturate_on/4(Tswh), Tgabc_on/1, Tgabc_off/2, Divide/1  "Tswh"
  Tgabc_off_h/1 -> Tgabc_on/2, Tgabc_off/1
  Tgabc_off/1 -> Demux1/1
  Tgabc_on/1 -> Demux/1
  Tabcs/1 -> Tgabc_off_h/1, Variant Subsystem/1(Tabc)
  Demux1/2 -> Saturate_on/2("Tgb_off ")
  Divide/1 -> Tabcs/1
  Constant6/1 -> Modulated/2
  Demux/1 -> Saturate_off/1("Tga_on ")
  Constant/1 -> Saturate_on/5(Tsw)
  Demux/2 -> Saturate_off/2("Tgb_on ")
  Demux1/3 -> Saturate_on/3("Tgc_off ")
  Demux1/1 -> Saturate_on/1("Tga_off ")
  Demux/3 -> Saturate_off/3("Tgc_on ")
  Saturate_off/3(Tgc_on) -> TON/3
  Saturate_off/1(Tga_on) -> TON/1
  TON/1 -> Add/2, TgabcON/1
  Saturate_off/2(Tgb_on) -> TON/2
  Saturate_on/3(Tgc_off) -> TOFF/3
  Saturate_on/1(Tga_off) -> TOFF/1
  Saturate_on/2(Tgb_off) -> TOFF/2
  TOFF/1 -> TgabcOFF/1, Add/1
  Add/1 -> Product3/1
  fsw/1 -> Product3/2  "Tsw"
  Product3/1 -> Modulated/1
  Modulated/1 -> Mod/1  "Modulated"

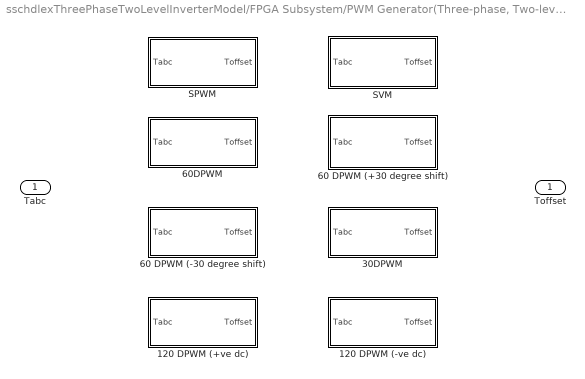
== system sschdlexThreePhaseTwoLevelInverterModel/FPGA Subsystem/PWM Generator(Three-phase, Two-level)/Switchingsignals/Variant Subsystem ==
  Tabc : Inport
  120 DPWM (+ve dc) : Subsystem  VariantControl=PWM==7
  120 DPWM (-ve dc) : Subsystem  VariantControl=PWM==8
  30DPWM : Subsystem  VariantControl=PWM==6
  60 DPWM (+30 degree shift) : Subsystem  VariantControl=PWM==4
  60 DPWM (-30 degree shift) : Subsystem  VariantControl=PWM==5
  60DPWM : Subsystem  VariantControl=PWM==3
  SPWM : Subsystem  VariantControl=PWM==1
  SVM : Subsystem  VariantControl=PWM==2
  Toffset : Outport

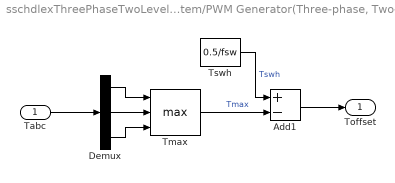
== system sschdlexThreePhaseTwoLevelInverterModel/FPGA Subsystem/PWM Generator(Three-phase, Two-level)/Switchingsignals/Variant Subsystem/120 DPWM (+ve dc) ==
  Tabc : Inport
  Add1 : Sum  Inputs=+-
  Demux : Demux  Outputs=3
  Tmax : MinMax  Function=max  Inputs=3  RndMeth=Simplest  OutDataTypeStr=Inherit: Same as first input
  Tswh : Constant  Value=0.5/fsw
  Toffset : Outport
  wires:
  Tmax/1 -> Add1/2  "Tmax"
  Demux/2 -> Tmax/2
  Demux/1 -> Tmax/1
  Tswh/1 -> Add1/1  "Tswh"
  Demux/3 -> Tmax/3
  Tabc/1 -> Demux/1
  Add1/1 -> Toffset/1

== system sschdlexThreePhaseTwoLevelInverterModel/FPGA Subsystem/PWM Generator(Three-phase, Two-level)/Switchingsignals/Variant Subsystem/120 DPWM (-ve dc) ==
  Tabc : Inport
  Constant : Constant  Value=-1  SampleTime=-1
  Demux : Demux  Outputs=3
  Product : Product
  Tmin : MinMax  Inputs=3  RndMeth=Simplest  OutDataTypeStr=Inherit: Same as first input
  Toffset : Outport
  wires:
  Constant/1 -> Product/2
  Demux/2 -> Tmin/2
  Tmin/1 -> Product/1  "Tmin"
  Demux/1 -> Tmin/1
  Demux/3 -> Tmin/3
  Product/1 -> Toffset/1
  Tabc/1 -> Demux/1

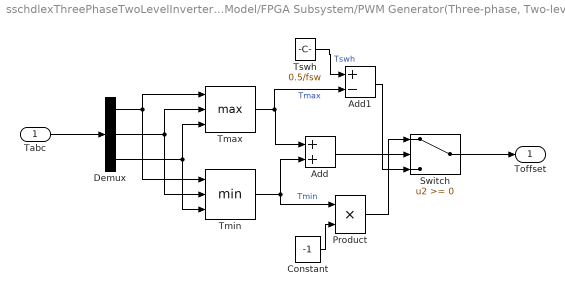
== system sschdlexThreePhaseTwoLevelInverterModel/FPGA Subsystem/PWM Generator(Three-phase, Two-level)/Switchingsignals/Variant Subsystem/30DPWM ==
  Tabc : Inport
  Add : Sum
  Add1 : Sum  Inputs=+-
  Constant : Constant  Value=-1  SampleTime=-1
  Demux : Demux  Outputs=3
  Product : Product
  Switch : Switch  SaturateOnIntegerOverflow=off  InputSameDT=off
  Tmax : MinMax  Function=max  Inputs=3  RndMeth=Simplest  OutDataTypeStr=Inherit: Same as first input
  Tmin : MinMax  Inputs=3  RndMeth=Simplest  OutDataTypeStr=Inherit: Same as first input
  Tswh : Constant  Value=0.5/fsw
  Toffset : Outport
  wires:
  Tabc/1 -> Demux/1
  Demux/3 -> Tmax/3, Tmin/3
  Demux/1 -> Tmax/1, Tmin/1
  Demux/2 -> Tmax/2, Tmin/2
  Tswh/1 -> Add1/1  "Tswh"
  Product/1 -> Switch/1
  Tmax/1 -> Add1/2, Add/1  "Tmax"
  Add/1 -> Switch/2
  Constant/1 -> Product/2
  Tmin/1 -> Product/1, Add/2  "Tmin"
  Add1/1 -> Switch/3
  Switch/1 -> Toffset/1

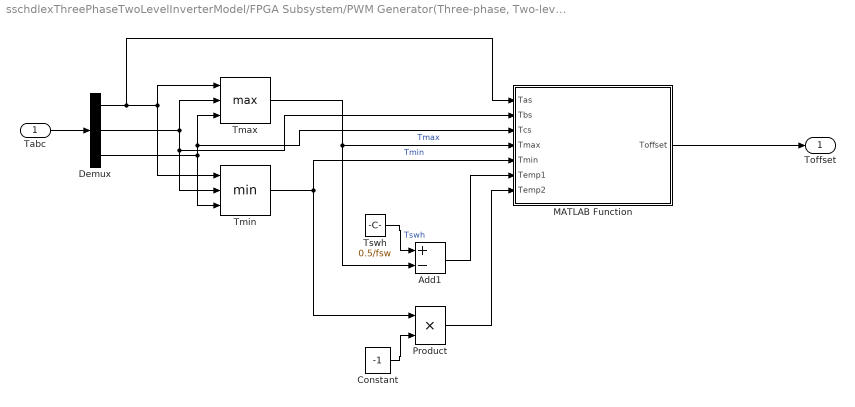
== system sschdlexThreePhaseTwoLevelInverterModel/FPGA Subsystem/PWM Generator(Three-phase, Two-level)/Switchingsignals/Variant Subsystem/60 DPWM (+30 degree shift) ==
  Tabc : Inport
  Add1 : Sum  Inputs=+-
  Constant : Constant  Value=-1  SampleTime=-1
  Demux : Demux  Outputs=3
  MATLAB Function : MATLAB Function  TreatAsAtomicUnit=on
  Product : Product
  Tmax : MinMax  Function=max  Inputs=3  RndMeth=Simplest  OutDataTypeStr=Inherit: Same as first input
  Tmin : MinMax  Inputs=3  RndMeth=Simplest  OutDataTypeStr=Inherit: Same as first input
  Tswh : Constant  Value=0.5/fsw
  Toffset : Outport
  wires:
  Tmax/1 -> MATLAB Function/4(Tmax), Add1/2  "Tmax"
  Constant/1 -> Product/2
  Tmin/1 -> MATLAB Function/5(Tmin), Product/1  "Tmin"
  Tswh/1 -> Add1/1  "Tswh"
  Demux/1 -> MATLAB Function/1(Tas), Tmax/1, Tmin/1
  Demux/3 -> MATLAB Function/3(Tcs), Tmax/3, Tmin/3
  Demux/2 -> MATLAB Function/2(Tbs), Tmin/2, Tmax/2
  Tabc/1 -> Demux/1
  Add1/1 -> MATLAB Function/6(Temp1)
  Product/1 -> MATLAB Function/7(Temp2)
  MATLAB Function/1(Toffset) -> Toffset/1

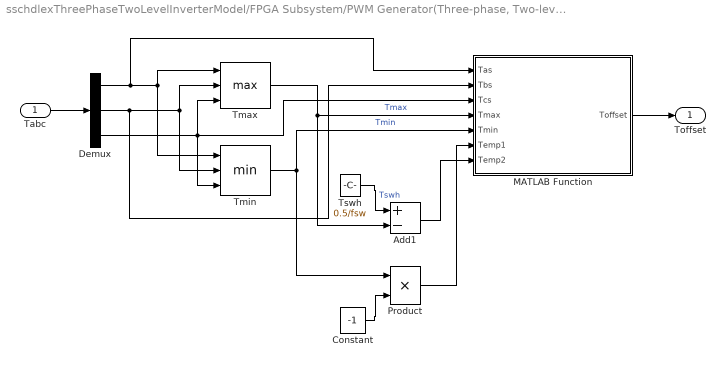
== system sschdlexThreePhaseTwoLevelInverterModel/FPGA Subsystem/PWM Generator(Three-phase, Two-level)/Switchingsignals/Variant Subsystem/60 DPWM (-30 degree shift) ==
  Tabc : Inport
  Add1 : Sum  Inputs=+-
  Constant : Constant  Value=-1  SampleTime=-1
  Demux : Demux  Outputs=3
  MATLAB Function : MATLAB Function  TreatAsAtomicUnit=on
  Product : Product
  Tmax : MinMax  Function=max  Inputs=3  RndMeth=Simplest  OutDataTypeStr=Inherit: Same as first input
  Tmin : MinMax  Inputs=3  RndMeth=Simplest  OutDataTypeStr=Inherit: Same as first input
  Tswh : Constant  Value=0.5/fsw
  Toffset : Outport
  wires:
  Tmax/1 -> MATLAB Function/4(Tmax), Add1/2  "Tmax"
  Demux/2 -> MATLAB Function/2(Tbs), Tmax/2, Tmin/2
  Tswh/1 -> Add1/1  "Tswh"
  Tabc/1 -> Demux/1
  Demux/1 -> MATLAB Function/1(Tas), Tmax/1, Tmin/1
  Demux/3 -> MATLAB Function/3(Tcs), Tmin/3, Tmax/3
  Constant/1 -> Product/2
  Tmin/1 -> Product/1, MATLAB Function/5(Tmin)  "Tmin"
  Product/1 -> MATLAB Function/6(Temp1)
  Add1/1 -> MATLAB Function/7(Temp2)
  MATLAB Function/1(Toffset) -> Toffset/1

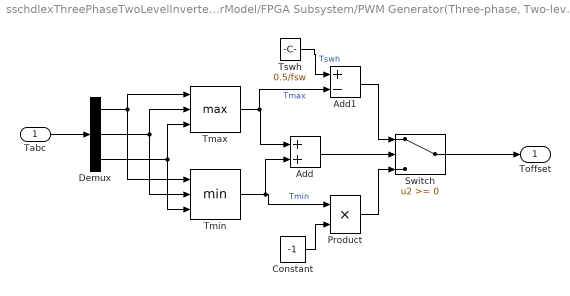
== system sschdlexThreePhaseTwoLevelInverterModel/FPGA Subsystem/PWM Generator(Three-phase, Two-level)/Switchingsignals/Variant Subsystem/60DPWM ==
  Tabc : Inport
  Add : Sum
  Add1 : Sum  Inputs=+-
  Constant : Constant  Value=-1  SampleTime=-1
  Demux : Demux  Outputs=3
  Product : Product
  Switch : Switch  SaturateOnIntegerOverflow=off  InputSameDT=off
  Tmax : MinMax  Function=max  Inputs=3  RndMeth=Simplest  OutDataTypeStr=Inherit: Same as first input
  Tmin : MinMax  Inputs=3  RndMeth=Simplest  OutDataTypeStr=Inherit: Same as first input
  Tswh : Constant  Value=0.5/fsw
  Toffset : Outport
  wires:
  Demux/3 -> Tmax/3, Tmin/3
  Demux/2 -> Tmax/2, Tmin/2
  Demux/1 -> Tmax/1, Tmin/1
  Tmax/1 -> Add1/2, Add/1  "Tmax"
  Tmin/1 -> Product/1, Add/2  "Tmin"
  Add/1 -> Switch/2
  Tswh/1 -> Add1/1  "Tswh"
  Add1/1 -> Switch/1
  Product/1 -> Switch/3
  Constant/1 -> Product/2
  Tabc/1 -> Demux/1
  Switch/1 -> Toffset/1

== system sschdlexThreePhaseTwoLevelInverterModel/FPGA Subsystem/PWM Generator(Three-phase, Two-level)/Switchingsignals/Variant Subsystem/SPWM ==
  Tabc : Inport
  Terminator : Terminator
  Tsw2 : Constant  Value=0.25/fsw
  Toffset : Outport
  wires:
  Tsw2/1 -> Toffset/1  "SPWM"
  Tabc/1 -> Terminator/1

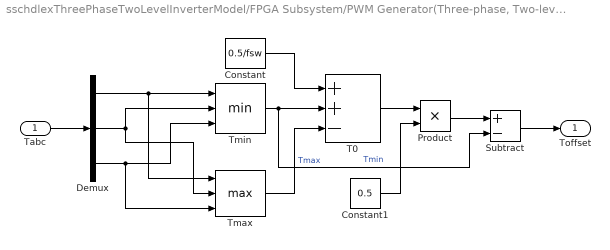
== system sschdlexThreePhaseTwoLevelInverterModel/FPGA Subsystem/PWM Generator(Three-phase, Two-level)/Switchingsignals/Variant Subsystem/SVM ==
  Tabc : Inport
  Constant : Constant  Value=0.5/fsw  SampleTime=-1
  Constant1 : Constant  Value=0.5  SampleTime=-1
  Demux : Demux  Outputs=3
  Product : Product
  Subtract : Sum  Inputs=+-
  T0 : Sum  Inputs=++-
  Tmax : MinMax  Function=max  Inputs=3  RndMeth=Simplest  OutDataTypeStr=Inherit: Same as first input
  Tmin : MinMax  Inputs=3  RndMeth=Simplest  OutDataTypeStr=Inherit: Same as first input
  Toffset : Outport
  wires:
  Tmin/1 -> T0/2, Subtract/2  "Tmin"
  Demux/2 -> Tmax/2, Tmin/2
  Tabc/1 -> Demux/1
  Tmax/1 -> T0/3  "Tmax"
  Constant/1 -> T0/1
  Demux/1 -> Tmax/1, Tmin/1
  Demux/3 -> Tmin/3, Tmax/3
  T0/1 -> Product/1
  Constant1/1 -> Product/2
  Product/1 -> Subtract/1
  Subtract/1 -> Toffset/1

== matlab function sschdlexThreePhaseTwoLevelInverterModel/FPGA Subsystem/PWM Generator(Three-phase, Two-level)/Switchingsignals/Saturate_off ==
  data: Tga_on input; Tga_on output; Tgb_on input; Tgc_on input; Tgb_on output; Tgc_on output; Tswh input
function [Tga_on,Tgb_on,Tgc_on] = Saturate_off(Tga_on,Tgb_on,Tgc_on,Tswh)
%#codegen
Tga_on = iSaturate(Tga_on,0,Tswh);
Tgb_on = iSaturate(Tgb_on,0,Tswh);
Tgc_on = iSaturate(Tgc_on,0,Tswh);
end
function x = iSaturate(x,xLowerLimit,xUpperLimit)
if x < xLowerLimit
    x = xLowerLimit;
elseif x > xUpperLimit
    x = xUpperLimit;
end
end

== matlab function sschdlexThreePhaseTwoLevelInverterModel/FPGA Subsystem/PWM Generator(Three-phase, Two-level)/Switchingsignals/Variant Subsystem/60 DPWM (-30 degree shift)/MATLAB Function ==
  data: Tas input; Toffset output; Tbs input; Tcs input; Tmax input; Tmin input; Temp1 input; Temp2 input
function Toffset = fcn(Tas, Tbs, Tcs, Tmax, Tmin, Temp1, Temp2)
Toffset=0;
if (((Tas == Tmax) && (Tcs == Tmin)) || ((Tbs == Tmax) && (Tas == Tmin)) || ((Tcs == Tmax) && (Tbs == Tmin)))
    Toffset = Temp1;
elseif (((Tbs == Tmax) && (Tcs == Tmin)) || ((Tcs == Tmax) && (Tas == Tmin)) || ((Tas == Tmax) && (Tbs == Tmin)))
    Toffset = Temp2;
end
end

== matlab function sschdlexThreePhaseTwoLevelInverterModel/FPGA Subsystem/PWM Generator(Three-phase, Two-level)/Switchingsignals/Saturate_on ==
  data: Tga_off input; Tga_off output; Tgb_off input; Tgc_off input; Tgb_off output; Tgc_off output; Tswh input; Tsw input
function [Tga_off,Tgb_off,Tgc_off] = Saturate_on(Tga_off,Tgb_off,Tgc_off,Tswh,Tsw)
%#codegen
Tga_off = iSaturate(Tga_off,Tswh,Tsw);
Tgb_off = iSaturate(Tgb_off,Tswh,Tsw);
Tgc_off = iSaturate(Tgc_off,Tswh,Tsw);
end
function x = iSaturate(x,xLowerLimit,xUpperLimit)
if x < xLowerLimit
    x = xLowerLimit;
elseif x > xUpperLimit
    x = xUpperLimit;
end
end

== matlab function sschdlexThreePhaseTwoLevelInverterModel/FPGA Subsystem/PWM Generator(Three-phase, Two-level)/Switchingsignals/Variant Subsystem/60 DPWM (+30 degree shift)/MATLAB Function ==
  data: Tas input; Toffset output; Tbs input; Tcs input; Tmax input; Tmin input; Temp1 input; Temp2 input
function Toffset = fcn(Tas, Tbs, Tcs, Tmax, Tmin, Temp1, Temp2)
Toffset=0;
if (((Tas == Tmax) && (Tcs == Tmin)) || ((Tbs == Tmax) && (Tas == Tmin)) || ((Tcs == Tmax) && (Tbs == Tmin)))
    Toffset = Temp1;
elseif (((Tbs == Tmax) && (Tcs == Tmin)) || ((Tcs == Tmax) && (Tas == Tmin)) || ((Tas == Tmax) && (Tbs == Tmin)))
    Toffset = Temp2;
end
end
